simulink model "power_measurements"  (R2026a)
settings: Solver=ode23tb  StopTime=simlength  FixedStep=tc  MaxStep=glb_time.tc
values from neighbouring files (symbols this model uses):
  glb_time = timing_setup(fpwm_afe, trgo_afe, fpwm_inv, trgo_inv, fpwm_single_phase_inv, trgo_single_phase_inv, fpwm_dab, trgo_dab,      fpwm_psfbc, trgo_psfbc, fpwm_isop_rail, trgo_isop_rail, fpwm_cllc, trgo_cllc, t_measure, tc_factor, tc_decimation, delay_pwm, dead_time_afe,      dead_time_inv, dead_time_single_phase_inv, dead_time_dab, dead_time_psfbc, dead_time_isop_rail, dead_time_cllc)    [init_model.m]
  grid_emu = grid_three_phase_emulator('Dyn11', delta_star, grid_nominal_power, application_voltage, us1, us2, fgrid,                  eq_grid_inductance, eq_grid_resistance, eta, ucc, i1m, p_iron, n1, n2, core_area, core_length, mur,                  up_xi_pu_ref, up_eta_pu_ref, un_xi_pu_ref, un_eta_pu_ref)    [init_model.m]
libraries: fl_lib x19, nesl_utility x16, single_phase_transformer_lib x3, three_phase_voltage_with_frt_emulator x1, power_meter_iec x1, three_phase_rl_load x1
settings Model: Creator=dbagn  LastModifiedBy=dbagn
settings SolverCC: NumberNewtonIterations=3.0  ZeroCrossControl=DisableAll  SolverResetMethod=Robust
settings SFSimCC: CustomCodeUndefinedFunction=ThrowError  DefaultCustomCodeDeterministicFunctions=All
settings SFSimCC: SimCustomHeaderCode=|
  | #include "rpi.h"
  | #include "rpi_simulink.h"
  | #include "bemf_obsv_load_est.h"
  | #include "bemf_obsv_load_est_simulink.h"
  | #include "dqpll_grid.h"
  | #include "dsmavgflt.h"
  | #include "bemf_obsv.h"
  | #include "bemf_obsv_simulink.h"
  | #include "mavgflt.h"
  | #include "mavgflt_simulink.h"
  | #include "mavgflts.h"
  | #include "mavgflts_simulink.h"
  | #include "sv_pwm_cm.h"
  | #include "dsmavgflt_simulink.h"
  | #include "linear_double_integrator_observer_simulink.h"
  | #include "sv_pwm_cm_simulink.h"
  | #include "dqvector_pi.h"
  | #include "dqpll_grid_simulink.h"
  | #include "first_harmonic_tracker.h"
  | #include "dqvector_pi_simulink.h"
  | #include "first_harmonic_tracker_simulink.h"
  | #include "dqpll_thyr.h"
  | #include "sv_pwm_simulink.h"
  | #include "sv_pwm.h"
  | #include "dqpll_thyr_simulink.h"
  | #include "linear_double_integrator_observer.h"
  | #include "math_f.h"
settings SFSimCC: SimUserSources=|
  | "rpi.c"
  | "rpi_simulink.c"
  | "mavgflt_simulink.c"
  | "mavgflt.c"
  | "mavgflts_simulink.c"
  | "mavgflts.c"
  | "dsmavgflt_simulink.c"
  | "dsmavgflt.c"
  | "bemf_obsv_simulink.c"
  | "bemf_obsv.c"
  | "bemf_obsv_load_est_simulink.c"
  | "bemf_obsv_load_est.c"
  | "dqvector_pi.c"
  | "dqvector_pi_simulink.c"
  | "sv_pwm_simulink.c"
  | "sv_pwm.c"
  | "first_harmonic_tracker_simulink.c"
  | "first_harmonic_tracker.c"
  | "dqpll_thyr_simulink.c"
  | "dqpll_thyr.c"
  | "dqpll_grid_simulink.c"
  | "dqpll_grid.c"
  | "linear_double_integrator_observer_simulink.c"
  | "linear_double_integrator_observer.c"
  | "sv_pwm_cm_simulink.c"
  | "sv_pwm_cm.c"
settings SFSimCC: SimUserIncludeDirs=|
  | include
  | src
settings SimscapeCC: SimscapeNominalValues="[{\"value\":\"1\",\"unit\":\"A\"},{\"value\":\"1\",\"unit\":\"bar\"},{\"value\":\"1\",\"unit\":\"cm^2\"},{\"value\":\"1\",\"unit\":\"cm^3/s\"},{\"value\":\"1\",\"unit\":\"kJ/kg\"},{\"value\":\"1\",\"unit\":\"kW\"},{\"value\":\"1\",\"unit\":\"l\"},{\"value\":\"1\",\"unit\":\"N\"},{\"value\":\"1\",\"unit\":\"N*m\"},{\"value\":\"1\",\"unit\":\"V\"}]"  SimscapeLogType=none  SimscapeLogDataHistory=5000.0

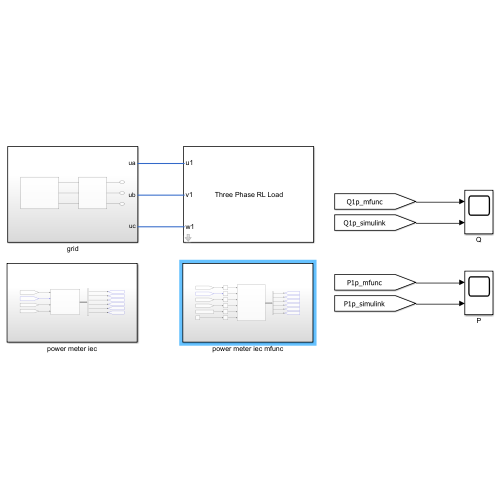
[thumbnail: Simulink's stored preview of the top-level diagram]
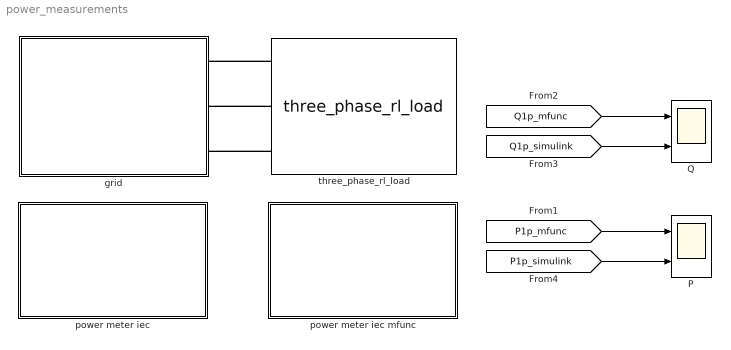
== system power_measurements ==
  P : Scope  NumInputPorts=2
      settings: ActiveDisplayYMinimum=-52907.922157185996  ActiveDisplayYMaximum=476171.29941467411
  Q : Scope  NumInputPorts=2
      settings: ActiveDisplayYMinimum=-16619.523856828953  ActiveDisplayYMaximum=149575.71471146061
  grid : Subsystem
  power meter iec : Subsystem
  power meter iec mfunc : Subsystem
  three_phase_rl_load : three_phase_rl_load/three_phase_rl_load  Ls_load=1e-3  Rs_load=1
  wires:
  [Q1p_mfunc] -> Q/1
  [Q1p_simulink] -> Q/2
  [P1p_mfunc] -> P/1
  [P1p_simulink] -> P/2
  connections:
  three_phase_rl_load/LConn1 -- grid/RConn1
  three_phase_rl_load/LConn3 -- grid/RConn3
  three_phase_rl_load/LConn2 -- grid/RConn2

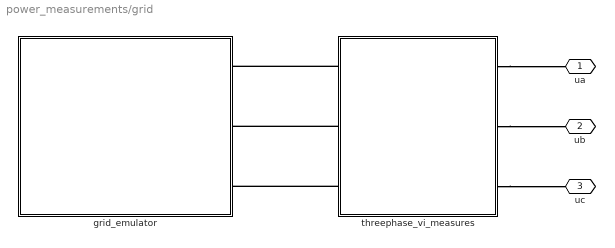
== system power_measurements/grid ==
  grid_emulator : Subsystem
  threephase_vi_measures : Subsystem
  ua : PMIOPort  Side=Right
  ub : PMIOPort  Port=2  Side=Right
  uc : PMIOPort  Port=3  Side=Right
  connections:
  threephase_vi_measures/LConn3 -- grid_emulator/RConn3
  threephase_vi_measures/LConn1 -- grid_emulator/RConn1
  threephase_vi_measures/RConn2 -- ub/RConn1
  threephase_vi_measures/LConn2 -- grid_emulator/RConn2
  threephase_vi_measures/RConn1 -- ua/RConn1
  threephase_vi_measures/RConn3 -- uc/RConn1

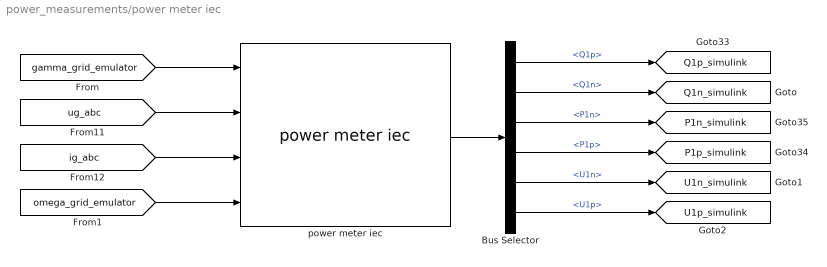
== system power_measurements/power meter iec ==
  Bus Selector : BusSelector  OutputSignals=Q1p,Q1n,P1n,P1p,U1n,U1p
  power meter iec : power_meter_iec/power meter iec  period=pi/grid_emu.omega_grid_nom  ts=glb_time.ts_afe  enable_time=0.025
  tag scope: P1n_simulink=global, P1p_simulink=global, Q1n_simulink=global, Q1p_simulink=global, U1n_simulink=global, U1p_simulink=global
  wires:
  power meter iec/1 -> Bus Selector/1
  Bus Selector/3 -> [P1n_simulink]  "<P1n>"
  [ug_abc] -> power meter iec/2
  [omega_grid_emulator] -> power meter iec/4
  Bus Selector/1 -> [Q1p_simulink]  "<Q1p>"
  Bus Selector/2 -> [Q1n_simulink]  "<Q1n>"
  Bus Selector/4 -> [P1p_simulink]  "<P1p>"
  [gamma_grid_emulator] -> power meter iec/1
  Bus Selector/5 -> [U1n_simulink]  "<U1n>"
  [ig_abc] -> power meter iec/3
  Bus Selector/6 -> [U1p_simulink]  "<U1p>"

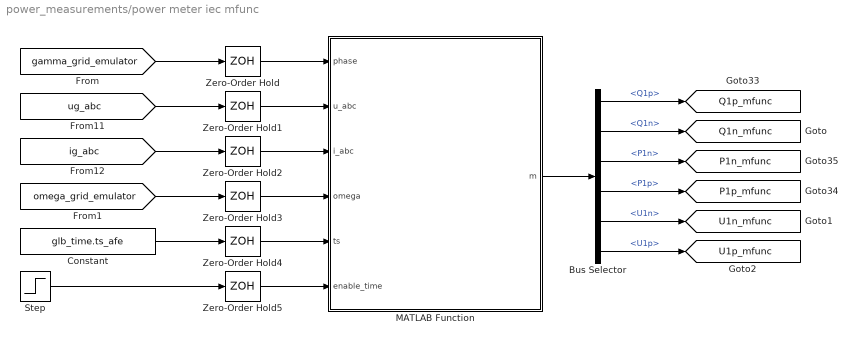
== system power_measurements/power meter iec mfunc ==
  Bus Selector : BusSelector  OutputSignals=Q1p,Q1n,P1n,P1p,U1n,U1p
  Constant : Constant  Value=glb_time.ts_afe
  MATLAB Function : MATLAB Function  TreatAsAtomicUnit=on  SystemSampleTime=glb_time.ts_afe
  Step : Step  Time=0.025  InitialValue=1  FinalValue=0  SampleTime=0
  Zero-Order Hold{,1..5} (6 alike) : ZeroOrderHold  SampleTime=glb_time.ts_afe
  tag scope: P1n_mfunc=global, P1p_mfunc=global, Q1n_mfunc=global, Q1p_mfunc=global, U1n_mfunc=global, U1p_mfunc=global
  wires:
  Bus Selector/6 -> [U1p_mfunc]  "<U1p>"
  [ig_abc] -> Zero-Order Hold2/1
  Bus Selector/5 -> [U1n_mfunc]  "<U1n>"
  [gamma_grid_emulator] -> Zero-Order Hold/1
  Bus Selector/4 -> [P1p_mfunc]  "<P1p>"
  Bus Selector/2 -> [Q1n_mfunc]  "<Q1n>"
  Bus Selector/1 -> [Q1p_mfunc]  "<Q1p>"
  [omega_grid_emulator] -> Zero-Order Hold3/1
  [ug_abc] -> Zero-Order Hold1/1
  Bus Selector/3 -> [P1n_mfunc]  "<P1n>"
  MATLAB Function/1(m) -> Bus Selector/1
  Constant/1 -> Zero-Order Hold4/1
  Step/1 -> Zero-Order Hold5/1
  Zero-Order Hold/1 -> MATLAB Function/1(phase)
  Zero-Order Hold1/1 -> MATLAB Function/2(u_abc)
  Zero-Order Hold2/1 -> MATLAB Function/3(i_abc)
  Zero-Order Hold3/1 -> MATLAB Function/4(omega)
  Zero-Order Hold4/1 -> MATLAB Function/5(ts)
  Zero-Order Hold5/1 -> MATLAB Function/6(enable_time)

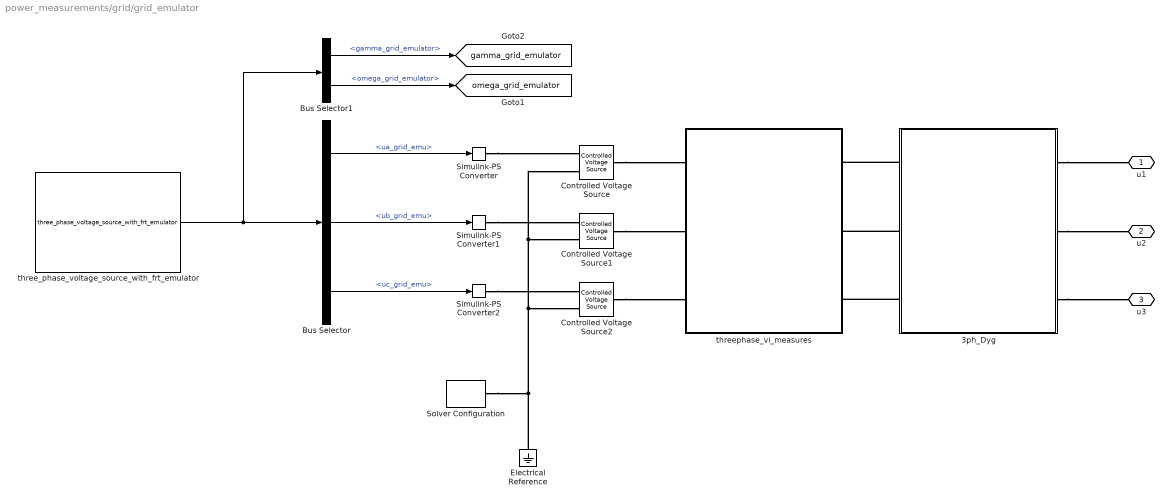
== system power_measurements/grid/grid_emulator ==
  3ph_Dyg : Subsystem
  Bus Selector : BusSelector  OutputSignals=ua_grid_emu,ub_grid_emu,uc_grid_emu
  Bus Selector1 : BusSelector  OutputSignals=gamma_grid_emulator,omega_grid_emulator
  Controlled Voltage Source : fl_lib/Electrical/Electrical Sources/Controlled Voltage Source
  Controlled Voltage Source1 : fl_lib/Electrical/Electrical Sources/Controlled Voltage Source
  Controlled Voltage Source2 : fl_lib/Electrical/Electrical Sources/Controlled Voltage Source
  Electrical Reference : fl_lib/Electrical/Electrical Elements/Electrical Reference
  Simulink-PS Converter : nesl_utility/Simulink-PS Converter  PhysicalDomain=network_engine_domain  SubClassName=ps_input  LeftPortType=input  RightPortType=output  PseudoPeriodic=off  Frequencies=[]  NoiseDistribution=none  NoiseParameters=[]  Unit=V  AffineConversion=on  FilteringAndDerivatives=provide  SimscapeFilterOrder=1  InputFilterTimeConstant=0.001  UdotUserProvided=0
  Simulink-PS Converter1 : nesl_utility/Simulink-PS Converter  PhysicalDomain=network_engine_domain  SubClassName=ps_input  LeftPortType=input  RightPortType=output  PseudoPeriodic=off  Frequencies=[]  NoiseDistribution=none  NoiseParameters=[]  Unit=V  AffineConversion=on  FilteringAndDerivatives=provide  SimscapeFilterOrder=1  InputFilterTimeConstant=0.001  UdotUserProvided=0
  Simulink-PS Converter2 : nesl_utility/Simulink-PS Converter  PhysicalDomain=network_engine_domain  SubClassName=ps_input  LeftPortType=input  RightPortType=output  PseudoPeriodic=off  Frequencies=[]  NoiseDistribution=none  NoiseParameters=[]  Unit=V  AffineConversion=on  FilteringAndDerivatives=provide  SimscapeFilterOrder=1  InputFilterTimeConstant=0.001  UdotUserProvided=0
  Solver Configuration : nesl_utility/Solver Configuration  PhysicalDomain=network_engine_domain  SubClassName=solver  LeftPortType=input  RightPortType=generic  Tones=[]  Harmonics=[]  SimulateNoise=off  Profile=off  UseLocalSampling=off  EnableSwitchedLinearOptims=on  FrequencyDomain=off  UseCCode=off  RelTol=0.001  AbsTol=0.001  MinStep=1e-09  ToWorkspace=off  RevertToSquareIcSolve=off  NumHomotopyIterations=100  PhasorMode=off  PhasorModeNumHarmonics=1  ConsistencySolver=NEWTON_FTOL  CanonicalOrdering=UNORDERED  OptimizeIntermediates=UNOPTIMIZED  IndexReductionMethod=DerivativeReplacement  DoDC=on  ResidualTolerance=1e-3  ConsistencyTolSource=GLOBAL  ConsistencyAbsTol=0.001  ConsistencyRelTol=0.001  ConsistencyTolFactor=0.001  UseLocalSolver=on  LocalSolverChoice=NE_BACKWARD_EULER_ADVANCER  ResolveIndetEquations=on  FunctionEvalNumThread=1  LocalSolverSampleTime=glb_time.tc  DoFixedCost=on  MaxNonlinIter=nonlinear_iterations  MaxModeIter=2  ComputeImpulses=off  ImpulseIterations=2  LinearAlgebra=auto  LinearAlgebraNumThread=0  EquationFormulation=NE_TIME_EF  DelaysMemoryBudget=1024  AutomaticFiltering=on  FilteringTimeConstant=0.001  PartitionStorageMethod=AS_NEEDED  PartitionMemoryBudget=1024  PartitionMethod=ROBUST  MultibodyUseLocalSolver=off  MultibodyLocalSolverChoice=ODE1  MultibodyLocalSolverSampleTime=0.001
  three_phase_voltage_source_with_frt_emulator : three_phase_voltage_with_frt_emulator/three_phase_voltage_source_with_frt_emulator  nominal_frequency_m=grid_emu.fgrid_nom  nominal_voltage_m=grid_emu.us_primary_nom  Vemu_ref_norm_m=grid_emu.Vemu_ref_norm  vp_xi_pu_m=grid_emu.up_xi_pu_ref  vp_eta_pu_m=grid_emu.up_eta_pu_ref  vn_xi_pu_m=grid_emu.un_xi_pu_ref  vn_eta_pu_m=grid_emu.un_eta_pu_ref  Am=filters.afe.SOF_50Hz.ss_c.A  Bm=filters.afe.SOF_50Hz.ss_c.B  Cm=filters.afe.SOF_50Hz.ss_c.C  enable_frt_1_m=frt_data.enable_frt_1  enable_frt_2_m=frt_data.enable_frt_2  start_time_LVRT_m=frt_data.start_time_LVRT  end_time_LVRT_m=frt_data.end_time_LVRT  deepPOSxi_m=frt_data.deepPOSxi  deepPOSeta_m=frt_data.deepPOSeta  deepNEGxi_m=frt_data.deepNEGxi  deepNEGeta_m=frt_data.deepNEGeta  Amplitude_U_m=frt_data.Amplitude_U  Amplitude_V_m=frt_data.Amplitude_V  Amplitude_W_m=frt_data.Amplitude_W  t_ramp_m=frt_data.t_ramp  Phase_shift_m=frt_data.Phase_shift
  threephase_vi_measures : Subsystem
  u1 : PMIOPort  Side=Right
  u2 : PMIOPort  Port=2  Side=Right
  u3 : PMIOPort  Port=3  Side=Right
  tag scope: gamma_grid_emulator=global, omega_grid_emulator=global
  wires:
  Bus Selector1/2 -> [omega_grid_emulator]  "<omega_grid_emulator>"
  Bus Selector1/1 -> [gamma_grid_emulator]  "<gamma_grid_emulator>"
  Bus Selector/2 -> Simulink-PS Converter1/1  "<ub_grid_emu>"
  Bus Selector/3 -> Simulink-PS Converter2/1  "<uc_grid_emu>"
  three_phase_voltage_source_with_frt_emulator/1 -> Bus Selector1/1, Bus Selector/1
  Bus Selector/1 -> Simulink-PS Converter/1  "<ua_grid_emu>"
  connections:
  Simulink-PS Converter/RConn1 -- Controlled Voltage Source/RConn1
  Simulink-PS Converter1/RConn1 -- Controlled Voltage Source1/RConn1
  Simulink-PS Converter2/RConn1 -- Controlled Voltage Source2/RConn1
  Electrical Reference/LConn1 -- Controlled Voltage Source/RConn2 -- Controlled Voltage Source1/RConn2 -- Controlled Voltage Source2/RConn2 -- Solver Configuration/RConn1
  3ph_Dyg/RConn1 -- u1/RConn1
  3ph_Dyg/RConn2 -- u2/RConn1
  3ph_Dyg/RConn3 -- u3/RConn1
  3ph_Dyg/LConn1 -- threephase_vi_measures/RConn1
  3ph_Dyg/LConn2 -- threephase_vi_measures/RConn2
  3ph_Dyg/LConn3 -- threephase_vi_measures/RConn3
  Controlled Voltage Source/LConn1 -- threephase_vi_measures/LConn1
  Controlled Voltage Source1/LConn1 -- threephase_vi_measures/LConn2
  Controlled Voltage Source2/LConn1 -- threephase_vi_measures/LConn3

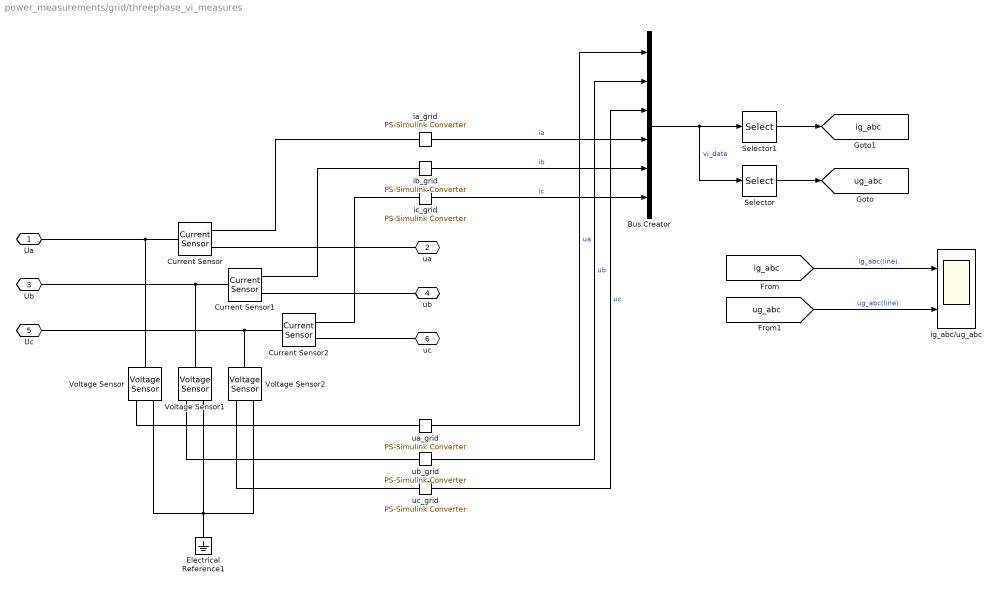
== system power_measurements/grid/threephase_vi_measures ==
  Bus Creator : BusCreator  Inputs=6
  Current Sensor : fl_lib/Electrical/Electrical Sensors/Current Sensor
  Current Sensor1 : fl_lib/Electrical/Electrical Sensors/Current Sensor
  Current Sensor2 : fl_lib/Electrical/Electrical Sensors/Current Sensor
  Electrical Reference1 : fl_lib/Electrical/Electrical Elements/Electrical Reference
  Selector : Selector  InputPortWidth=6  IndexOptions=Index vector (dialog)  Indices=[1 2 3]  OutputSizes=1
  Selector1 : Selector  InputPortWidth=6  IndexOptions=Index vector (dialog)  Indices=[4 5 6]  OutputSizes=1
  Voltage Sensor : fl_lib/Electrical/Electrical Sensors/Voltage Sensor
  Voltage Sensor1 : fl_lib/Electrical/Electrical Sensors/Voltage Sensor
  Voltage Sensor2 : fl_lib/Electrical/Electrical Sensors/Voltage Sensor
  ia_grid : nesl_utility/PS-Simulink Converter  PhysicalDomain=network_engine_domain  SubClassName=ps_output  LeftPortType=input  RightPortType=output  PseudoPeriodic=off  Frequencies=[]  VectorFormat=1-D array  Unit=A  AffineConversion=off
  ib_grid : nesl_utility/PS-Simulink Converter  PhysicalDomain=network_engine_domain  SubClassName=ps_output  LeftPortType=input  RightPortType=output  PseudoPeriodic=off  Frequencies=[]  VectorFormat=1-D array  Unit=A  AffineConversion=off
  ic_grid : nesl_utility/PS-Simulink Converter  PhysicalDomain=network_engine_domain  SubClassName=ps_output  LeftPortType=input  RightPortType=output  PseudoPeriodic=off  Frequencies=[]  VectorFormat=1-D array  Unit=A  AffineConversion=off
  ig_abc/ug_abc : Scope  NumInputPorts=2
      settings: SampleTime=glb_time.tc  ActiveDisplayYMinimum=-728.92703752654245  ActiveDisplayYMaximum=734.90808013997  DataLoggingVariableName=ScopeData2
  ua_grid : nesl_utility/PS-Simulink Converter  PhysicalDomain=network_engine_domain  SubClassName=ps_output  LeftPortType=input  RightPortType=output  PseudoPeriodic=off  Frequencies=[]  VectorFormat=1-D array  Unit=V  AffineConversion=off
  ub_grid : nesl_utility/PS-Simulink Converter  PhysicalDomain=network_engine_domain  SubClassName=ps_output  LeftPortType=input  RightPortType=output  PseudoPeriodic=off  Frequencies=[]  VectorFormat=1-D array  Unit=V  AffineConversion=off
  uc_grid : nesl_utility/PS-Simulink Converter  PhysicalDomain=network_engine_domain  SubClassName=ps_output  LeftPortType=input  RightPortType=output  PseudoPeriodic=off  Frequencies=[]  VectorFormat=1-D array  Unit=V  AffineConversion=off
  Ua : PMIOPort  Side=Left
  ua : PMIOPort  Port=2  Side=Right
  Ub : PMIOPort  Port=3  Side=Left
  ub : PMIOPort  Port=4  Side=Right
  Uc : PMIOPort  Port=5  Side=Left
  uc : PMIOPort  Port=6  Side=Right
  tag scope: ig_abc=global, ug_abc=global
  wires:
  Bus Creator/1 -> Selector1/1, Selector/1  "vi_data"
  Selector/1 -> [ug_abc]
  ib_grid/1 -> Bus Creator/5  "ib"
  ia_grid/1 -> Bus Creator/4  "ia"
  ic_grid/1 -> Bus Creator/6  "ic"
  ua_grid/1 -> Bus Creator/1  "ua"
  ub_grid/1 -> Bus Creator/2  "ub"
  uc_grid/1 -> Bus Creator/3  "uc"
  Selector1/1 -> [ig_abc]
  [ug_abc] -> ig_abc/ug_abc/2  "ug_abc(line)"
  [ig_abc] -> ig_abc/ug_abc/1  "ig_abc(line)"
  connections:
  Current Sensor1/LConn1 -- Ub/RConn1 -- Voltage Sensor1/LConn1
  Electrical Reference1/LConn1 -- Voltage Sensor/RConn2 -- Voltage Sensor2/RConn2 -- Voltage Sensor1/RConn2
  Voltage Sensor/RConn1 -- ua_grid/LConn1
  Current Sensor/RConn2 -- ua/RConn1
  Voltage Sensor1/RConn1 -- ub_grid/LConn1
  Voltage Sensor2/LConn1 -- Current Sensor2/LConn1 -- Uc/RConn1
  Current Sensor/LConn1 -- Ua/RConn1 -- Voltage Sensor/LConn1
  Current Sensor1/RConn2 -- ub/RConn1
  Voltage Sensor2/RConn1 -- uc_grid/LConn1
  ib_grid/LConn1 -- Current Sensor1/RConn1
  ia_grid/LConn1 -- Current Sensor/RConn1
  ic_grid/LConn1 -- Current Sensor2/RConn1
  Current Sensor2/RConn2 -- uc/RConn1

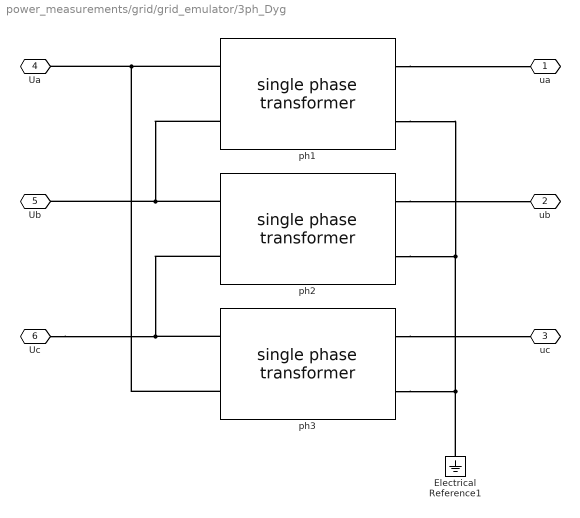
== system power_measurements/grid/grid_emulator/3ph_Dyg ==
  Electrical Reference1 : fl_lib/Electrical/Electrical Elements/Electrical Reference
  ph1 : single_phase_transformer_lib/single phase transformer  Lm=grid_emu.trafo.Lm1 H  n1=grid_emu.trafo.n1  n2=grid_emu.trafo.n2  Rd1=grid_emu.trafo.Rd1 Ohm  Rd2=grid_emu.trafo.Rd2 Ohm  Ld1=grid_emu.trafo.Ld1 H  Ld2=grid_emu.trafo.Ld2 H  Rfe=grid_emu.trafo.Rfe1 Ohm  phi_specify=off  phi_priority=None  phi=0 V*s  phi_nominal_specify=off  phi_nominal_value=1  phi_nominal_unit=V*s  i1_specify=off  i1_priority=None  i1=0 A  i1_nominal_specify=off  i1_nominal_value=1  i1_nominal_unit=A  i2_specify=off  i2_priority=None  i2=0 A  i2_nominal_specify=off  i2_nominal_value=1  i2_nominal_unit=A  ife_specify=off  ife_priority=None  ife=0 A  ife_nominal_specify=off  ife_nominal_value=1  ife_nominal_unit=A  u1_specify=off  u1_priority=None  u1=0 V  u1_nominal_specify=off  u1_nominal_value=1  u1_nominal_unit=V  u2_specify=off  u2_priority=None  u2=0 V  u2_nominal_specify=off  u2_nominal_value=1  u2_nominal_unit=V
  ph2 : single_phase_transformer_lib/single phase transformer  Lm=grid_emu.trafo.Lm1 H  n1=grid_emu.trafo.n1  n2=grid_emu.trafo.n2  Rd1=grid_emu.trafo.Rd1 Ohm  Rd2=grid_emu.trafo.Rd2 Ohm  Ld1=grid_emu.trafo.Ld1 H  Ld2=grid_emu.trafo.Ld2 H  Rfe=grid_emu.trafo.Rfe1 Ohm  phi_specify=off  phi_priority=None  phi=0 V*s  phi_nominal_specify=off  phi_nominal_value=1  phi_nominal_unit=V*s  i1_specify=off  i1_priority=None  i1=0 A  i1_nominal_specify=off  i1_nominal_value=1  i1_nominal_unit=A  i2_specify=off  i2_priority=None  i2=0 A  i2_nominal_specify=off  i2_nominal_value=1  i2_nominal_unit=A  ife_specify=off  ife_priority=None  ife=0 A  ife_nominal_specify=off  ife_nominal_value=1  ife_nominal_unit=A  u1_specify=off  u1_priority=None  u1=0 V  u1_nominal_specify=off  u1_nominal_value=1  u1_nominal_unit=V  u2_specify=off  u2_priority=None  u2=0 V  u2_nominal_specify=off  u2_nominal_value=1  u2_nominal_unit=V
  ph3 : single_phase_transformer_lib/single phase transformer  Lm=grid_emu.trafo.Lm1 H  n1=grid_emu.trafo.n1  n2=grid_emu.trafo.n2  Rd1=grid_emu.trafo.Rd1 Ohm  Rd2=grid_emu.trafo.Rd2 Ohm  Ld1=grid_emu.trafo.Ld1 H  Ld2=grid_emu.trafo.Ld2 H  Rfe=grid_emu.trafo.Rfe1 Ohm  phi_specify=off  phi_priority=None  phi=0 V*s  phi_nominal_specify=off  phi_nominal_value=1  phi_nominal_unit=V*s  i1_specify=off  i1_priority=None  i1=0 A  i1_nominal_specify=off  i1_nominal_value=1  i1_nominal_unit=A  i2_specify=off  i2_priority=None  i2=0 A  i2_nominal_specify=off  i2_nominal_value=1  i2_nominal_unit=A  ife_specify=off  ife_priority=None  ife=0 A  ife_nominal_specify=off  ife_nominal_value=1  ife_nominal_unit=A  u1_specify=off  u1_priority=None  u1=0 V  u1_nominal_specify=off  u1_nominal_value=1  u1_nominal_unit=V  u2_specify=off  u2_priority=None  u2=0 V  u2_nominal_specify=off  u2_nominal_value=1  u2_nominal_unit=V
  ua : PMIOPort  Side=Right
  ub : PMIOPort  Port=2  Side=Right
  uc : PMIOPort  Port=3  Side=Right
  Ua : PMIOPort  Port=4  Side=Left
  Ub : PMIOPort  Port=5  Side=Left
  Uc : PMIOPort  Port=6  Side=Left
  connections:
  Electrical Reference1/LConn1 -- ph3/RConn2 -- ph2/RConn2 -- ph1/RConn2
  ph3/RConn1 -- uc/RConn1
  ph1/LConn1 -- ph3/LConn2 -- Ua/RConn1
  ph1/RConn1 -- ua/RConn1
  ph2/RConn1 -- ub/RConn1
  ph1/LConn2 -- ph2/LConn1 -- Ub/RConn1
  Uc/RConn1 -- ph3/LConn1 -- ph2/LConn2

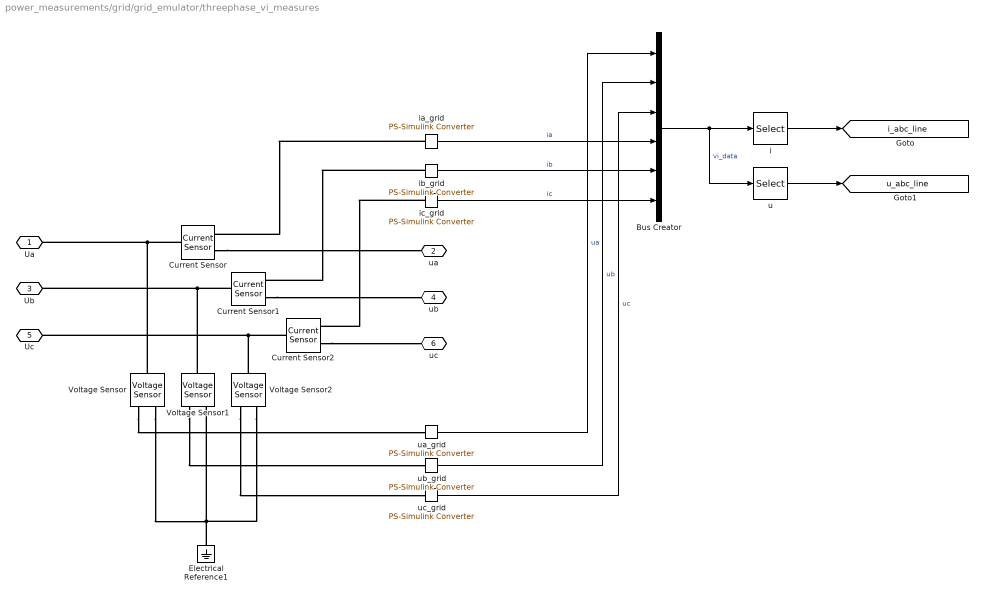
== system power_measurements/grid/grid_emulator/threephase_vi_measures ==
  Bus Creator : BusCreator  Inputs=6
  Current Sensor : fl_lib/Electrical/Electrical Sensors/Current Sensor
  Current Sensor1 : fl_lib/Electrical/Electrical Sensors/Current Sensor
  Current Sensor2 : fl_lib/Electrical/Electrical Sensors/Current Sensor
  Electrical Reference1 : fl_lib/Electrical/Electrical Elements/Electrical Reference
  Voltage Sensor : fl_lib/Electrical/Electrical Sensors/Voltage Sensor
  Voltage Sensor1 : fl_lib/Electrical/Electrical Sensors/Voltage Sensor
  Voltage Sensor2 : fl_lib/Electrical/Electrical Sensors/Voltage Sensor
  i : Selector  InputPortWidth=6  IndexOptions=Index vector (dialog)  Indices=[4 5 6]  OutputSizes=1
  ia_grid : nesl_utility/PS-Simulink Converter  PhysicalDomain=network_engine_domain  SubClassName=ps_output  LeftPortType=input  RightPortType=output  PseudoPeriodic=off  Frequencies=[]  VectorFormat=1-D array  Unit=A  AffineConversion=off
  ib_grid : nesl_utility/PS-Simulink Converter  PhysicalDomain=network_engine_domain  SubClassName=ps_output  LeftPortType=input  RightPortType=output  PseudoPeriodic=off  Frequencies=[]  VectorFormat=1-D array  Unit=A  AffineConversion=off
  ic_grid : nesl_utility/PS-Simulink Converter  PhysicalDomain=network_engine_domain  SubClassName=ps_output  LeftPortType=input  RightPortType=output  PseudoPeriodic=off  Frequencies=[]  VectorFormat=1-D array  Unit=A  AffineConversion=off
  u : Selector  InputPortWidth=6  IndexOptions=Index vector (dialog)  Indices=[1 2 3]  OutputSizes=1
  ua_grid : nesl_utility/PS-Simulink Converter  PhysicalDomain=network_engine_domain  SubClassName=ps_output  LeftPortType=input  RightPortType=output  PseudoPeriodic=off  Frequencies=[]  VectorFormat=1-D array  Unit=V  AffineConversion=off
  ub_grid : nesl_utility/PS-Simulink Converter  PhysicalDomain=network_engine_domain  SubClassName=ps_output  LeftPortType=input  RightPortType=output  PseudoPeriodic=off  Frequencies=[]  VectorFormat=1-D array  Unit=V  AffineConversion=off
  uc_grid : nesl_utility/PS-Simulink Converter  PhysicalDomain=network_engine_domain  SubClassName=ps_output  LeftPortType=input  RightPortType=output  PseudoPeriodic=off  Frequencies=[]  VectorFormat=1-D array  Unit=V  AffineConversion=off
  Ua : PMIOPort  Side=Left
  ua : PMIOPort  Port=2  Side=Right
  Ub : PMIOPort  Port=3  Side=Left
  ub : PMIOPort  Port=4  Side=Right
  Uc : PMIOPort  Port=5  Side=Left
  uc : PMIOPort  Port=6  Side=Right
  tag scope: i_abc_line=global, u_abc_line=global
  wires:
  Bus Creator/1 -> i/1, u/1  "vi_data"
  ib_grid/1 -> Bus Creator/5  "ib"
  ia_grid/1 -> Bus Creator/4  "ia"
  ic_grid/1 -> Bus Creator/6  "ic"
  ua_grid/1 -> Bus Creator/1  "ua"
  ub_grid/1 -> Bus Creator/2  "ub"
  uc_grid/1 -> Bus Creator/3  "uc"
  i/1 -> [i_abc_line]
  u/1 -> [u_abc_line]
  connections:
  Current Sensor1/LConn1 -- Ub/RConn1 -- Voltage Sensor1/LConn1
  Electrical Reference1/LConn1 -- Voltage Sensor/RConn2 -- Voltage Sensor2/RConn2 -- Voltage Sensor1/RConn2
  Voltage Sensor/RConn1 -- ua_grid/LConn1
  Current Sensor/RConn2 -- ua/RConn1
  Voltage Sensor1/RConn1 -- ub_grid/LConn1
  Voltage Sensor2/LConn1 -- Current Sensor2/LConn1 -- Uc/RConn1
  Current Sensor/LConn1 -- Ua/RConn1 -- Voltage Sensor/LConn1
  Current Sensor1/RConn2 -- ub/RConn1
  Voltage Sensor2/RConn1 -- uc_grid/LConn1
  ib_grid/LConn1 -- Current Sensor1/RConn1
  ia_grid/LConn1 -- Current Sensor/RConn1
  ic_grid/LConn1 -- Current Sensor2/RConn1
  Current Sensor2/RConn2 -- uc/RConn1

== matlab function power_measurements/power meter iec mfunc/MATLAB Function ==
  data: phase input; m output Bus: PowerMeterIecBus; u_abc input; i_abc input; omega input; ts input; enable_time input
function m = three_phase_power_meter_iec(phase, u_abc, i_abc, omega, ts, enable_time)
%#codegen
% THREE_PHASE_POWER_METER_IEC
% Equivalente in singolo blocco MATLAB Function del sottosistema Simulink
% "three_phase_power_meter_iec" (libreria power_meter_iec).
%
% INGRESSI
%   phase       : angolo del PLL [rad]      (scalare)
%   u_abc       : tensioni di fase [V]      (3x1)
%   i_abc       : correnti di linea [A]     (3x1)
%   omega       : pulsazione di rete [rad/s] (scalare)
%   ts          : passo di campionamento [s]  -> parametro di maschera
%   enable_time : istante di abilitazione [s] -> parametro di maschera
%
% USCITA
%   m : struct (bus) con i campi, nello stesso ordine del Bus Creator
%       originale: Q1p, Q1n, P1n, P1p, U1n, U1p,
%                  i_act_1n, i_react_1n, i_act_1p, i_react_1p
%
% CATENA DI ELABORAZIONE (identica all'originale)
%   1) proiezione di ogni fase su cos(phase) e sin(phase), guadagno 2
%   2) media mobile dinamica su finestra pari a mezzo periodo di rete
%      (Tw = pi/|omega|), con lunghezza frazionaria interpolata
%   3) componenti simmetriche di sequenza diretta e inversa (Fortescue)
%   4) potenze attiva e reattiva per sequenza, tensioni concatenate RMS,
%      correnti attiva e reattiva per sequenza
%
% NOTE
%   - Il blocco deve girare a passo fisso ts (gli Zero-Order Hold di
%     ingresso dell'originale sono impliciti nel sample time del blocco).
%   - ts ed enable_time possono essere dichiarati come dati di scope
%     "Parameter" nel Symbols pane del MATLAB Function block, cosi'
%     risolvono direttamente sui parametri di maschera e la firma
%     esterna resta a 4 ingressi come nel blocco originale.

% ------------------------------------------------------------------
% Costanti
% ------------------------------------------------------------------
MAVGFLT_SIZE_MAX = 17500;   % lunghezza buffer circolare (come originale)
NCH              = 12;      % canali filtrati: 6 per u_abc, 6 per i_abc

% Ordine canali:
%   1..3  ua_cos ub_cos uc_cos      7..9   ia_cos ib_cos ic_cos
%   4..6  ua_sin ub_sin uc_sin     10..12  ia_sin ib_sin ic_sin

% ------------------------------------------------------------------
% Stato persistente
% ------------------------------------------------------------------
persistent buf cb_index sample_count sum_short sum_long prev_input ...
           k_step period_held

if isempty(buf)
    buf          = zeros(NCH, MAVGFLT_SIZE_MAX);
    cb_index     = ones(NCH, 1);
    sample_count = ones(NCH, 1);
    sum_short    = zeros(NCH, 1);
    sum_long     = zeros(NCH, 1);
    prev_input   = zeros(NCH, 1);
    k_step       = 0;
    period_held  = 0;          % uscita iniziale dell'Enabled Subsystem
end

% ------------------------------------------------------------------
% Abilitazione (equivalente al blocco Step con Time = enable_time)
% ------------------------------------------------------------------
t_now  = k_step * ts;
k_step = k_step + 1;
enable = (t_now >= enable_time);

% ------------------------------------------------------------------
% Finestra di media: Enabled Subsystem 2*pi/w, alimentato da 2*|omega|.
% Quando |omega| = 0 l'Enabled Subsystem mantiene l'ultimo valore.
% ------------------------------------------------------------------
w2 = 2 * abs(omega);
if w2 > 0
    period_held = 2*pi / w2;   % = pi/|omega|, mezzo periodo di rete
end
period = period_held;

% ------------------------------------------------------------------
% Proiezione sin/cos, guadagno 2
% ------------------------------------------------------------------
c = cos(phase);
s = sin(phase);

x = zeros(NCH, 1);
x(1)  = 2 * u_abc(1) * c;   x(2)  = 2 * u_abc(2) * c;   x(3)  = 2 * u_abc(3) * c;
x(4)  = 2 * u_abc(1) * s;   x(5)  = 2 * u_abc(2) * s;   x(6)  = 2 * u_abc(3) * s;
x(7)  = 2 * i_abc(1) * c;   x(8)  = 2 * i_abc(2) * c;   x(9)  = 2 * i_abc(3) * c;
x(10) = 2 * i_abc(1) * s;   x(11) = 2 * i_abc(2) * s;   x(12) = 2 * i_abc(3) * s;

% ------------------------------------------------------------------
% Banco di 12 filtri a media mobile dinamica (dmavgflt_process)
% ------------------------------------------------------------------
y = zeros(NCH, 1);

if enable && period > 0

    desired = period / ts;
    if desired > (MAVGFLT_SIZE_MAX - 1)
        desired = MAVGFLT_SIZE_MAX - 1;
    end

    n_samples = floor(desired + 1);          % campioni che coprono il periodo
    frac      = desired + 1 - n_samples;     % parte frazionaria
    if n_samples < 1
        n_samples = 1;
    end

    for ch = 1:NCH

        ci = cb_index(ch);
        sc = sample_count(ch);

        if n_samples > sc
            % finestra in crescita: aggiungi campioni
            sum_short(ch) = sum_short(ch) + prev_input(ch);
            sum_long(ch)  = sum_long(ch)  + x(ch);
            sc = sc + 1;

        elseif n_samples < sc
            % finestra in contrazione: rimuovi i due campioni piu' vecchi
            i1 = mod(ci - 1 - sc,       MAVGFLT_SIZE_MAX) + 1;
            i2 = mod(ci - 1 - (sc - 1), MAVGFLT_SIZE_MAX) + 1;
            old_sum = buf(ch, i1) + buf(ch, i2);

            sum_short(ch) = sum_short(ch) + prev_input(ch) - old_sum;
            sum_long(ch)  = sum_long(ch)  + x(ch)          - old_sum;
            sc = sc - 1;

        else
            % finestra costante
            i1     = mod(ci - 1 - sc, MAVGFLT_SIZE_MAX) + 1;
            oldest = buf(ch, i1);

            sum_short(ch) = sum_short(ch) + prev_input(ch) - oldest;
            sum_long(ch)  = sum_long(ch)  + x(ch)          - oldest;
        end

        % aggiornamento buffer circolare
        buf(ch, ci)      = x(ch);
        cb_index(ch)     = mod(ci, MAVGFLT_SIZE_MAX) + 1;
        prev_input(ch)   = x(ch);
        sample_count(ch) = sc;

        % uscita: interpolazione lineare fra finestra corta e lunga
        if sc > 1
            avg_short = sum_short(ch) / (sc - 1);
        else
            avg_short = 0;
        end
        avg_long = sum_long(ch) / sc;

        y(ch) = avg_short * (1 - frac) + avg_long * frac;
    end
end
% se enable = false oppure period <= 0: y resta 0 e lo stato non evolve
% (comportamento identico all'originale)

ua_cos = y(1);  ub_cos = y(2);  uc_cos = y(3);
ua_sin = y(4);  ub_sin = y(5);  uc_sin = y(6);
ia_cos = y(7);  ib_cos = y(8);  ic_cos = y(9);
ia_sin = y(10); ib_sin = y(11); ic_sin = y(12);

% ------------------------------------------------------------------
% Componenti simmetriche (fasori con convenzione U = u_cos - j*u_sin)
% ------------------------------------------------------------------
sq3 = sqrt(3);

u1p_cos = (2*ua_cos - ub_cos - uc_cos - sq3*(uc_sin - ub_sin)) / 6;
u1p_sin = (2*ua_sin - ub_sin - uc_sin - sq3*(ub_cos - uc_cos)) / 6;
u1n_cos = (2*ua_cos - ub_cos - uc_cos - sq3*(ub_sin - uc_sin)) / 6;
u1n_sin = (2*ua_sin - ub_sin - uc_sin - sq3*(uc_cos - ub_cos)) / 6;

i1p_cos = (2*ia_cos - ib_cos - ic_cos - sq3*(ic_sin - ib_sin)) / 6;
i1p_sin = (2*ia_sin - ib_sin - ic_sin - sq3*(ib_cos - ic_cos)) / 6;
i1n_cos = (2*ia_cos - ib_cos - ic_cos - sq3*(ib_sin - ic_sin)) / 6;
i1n_sin = (2*ia_sin - ib_sin - ic_sin - sq3*(ic_cos - ib_cos)) / 6;

% ------------------------------------------------------------------
% Potenze per sequenza
% ------------------------------------------------------------------
P1p = 1.5 * (u1p_cos*i1p_cos + u1p_sin*i1p_sin);
Q1p = 1.5 * (u1p_cos*i1p_sin - u1p_sin*i1p_cos);
P1n = 1.5 * (u1n_cos*i1n_cos + u1n_sin*i1n_sin);
Q1n = 1.5 * (u1n_cos*i1n_sin - u1n_sin*i1n_cos);

% ------------------------------------------------------------------
% Tensioni concatenate RMS per sequenza: sqrt(3/2)*ampiezza di fase
% ------------------------------------------------------------------
U1p = sqrt(1.5 * (u1p_cos^2 + u1p_sin^2));
U1n = sqrt(1.5 * (u1n_cos^2 + u1n_sin^2));

% ------------------------------------------------------------------
% Correnti attiva e reattiva per sequenza (RMS di linea)
% La protezione contro la divisione per zero non era presente nello
% schema originale (i blocchi Divide restituivano Inf/NaN a U = 0).
% Portare U_MIN a 0 per replicare esattamente il comportamento vecchio.
% ------------------------------------------------------------------
U_MIN = 1e-9;

if U1p > U_MIN
    i_act_1p   = P1p / (sq3 * U1p);
    i_react_1p = Q1p / (sq3 * U1p);
else
    i_act_1p   = 0;
    i_react_1p = 0;
end

if U1n > U_MIN
    i_act_1n   = P1n / (sq3 * U1n);
    i_react_1n = Q1n / (sq3 * U1n);
else
    i_act_1n   = 0;
    i_react_1n = 0;
end

% ------------------------------------------------------------------
% Bus di uscita (stesso ordine dei campi dell'originale)
% ------------------------------------------------------------------
m.Q1p        = Q1p;
m.Q1n        = Q1n;
m.P1n        = P1n;
m.P1p        = P1p;
m.U1n        = U1n;
m.U1p        = U1p;
m.i_act_1n   = i_act_1n;
m.i_react_1n = i_react_1n;
m.i_act_1p   = i_act_1p;
m.i_react_1p = i_react_1p;

end
